simulink model "quadrotor_1d_v3"  (R2025b)
settings: Solver=ode45  StartTime=0.0  StopTime=20  MaxStep=0.005  RelTol=1e-3
values from neighbouring files (symbols this model uses):
  agr_scale = 1.4    [quad_params_v2.m]
  c_d = 0.1    [quad_params_v2.m]
  ctrl_mode = 0    [quad_params_v2.m]    (also in run_compare_v2.m)
  g = 9.81    [quad_params_v2.m]
  gamma = 0.40    (= 0.4)    [quad_params_v2.m]
  k_f = m*g/(4*w_hover^2)    (= 5.00510204082e-06)    [quad_params_v2.m]
  Kd0 = Kd    [design_pid_v2.m]
  Ki0 = Ki    [design_pid_v2.m]
  Kp0 = Kp    [design_pid_v2.m]
  m = 1.0    (= 1)    [quad_params_v2.m]
  tau_m = 0.05    [quad_params_v2.m]
  U_max = 2*m*g    (= 19.62)    [quad_params_v2.m]
  w_hover = 700    [quad_params_v2.m]
  w_max = sqrt(U_max/(4*k_f))    [quad_params_v2.m]
  wind_amp = -6.0    (= -6)    [quad_params_v2.m]
  wind_dur = 3.0    (= 3)    [quad_params_v2.m]
  wind_t0 = 5.0    (= 5)    [quad_params_v2.m]
  z0 = 0    [quad_params_v2.m]
undefined symbols (not defined in the file or in its folder): b1, b2, b3, W1, W2, W3
libraries: simulink x2
settings Model: Creator=Monster  LastModifiedBy=Monster

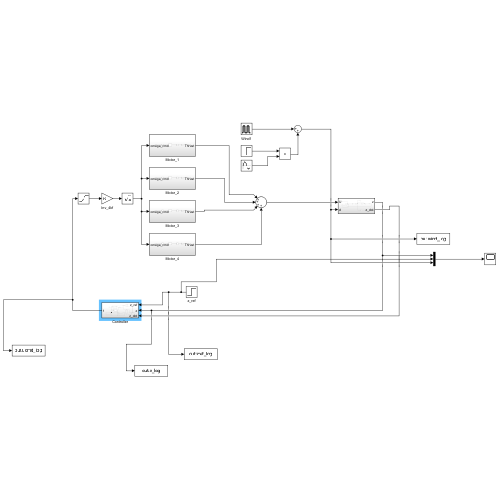
[thumbnail: Simulink's stored preview of the top-level diagram]
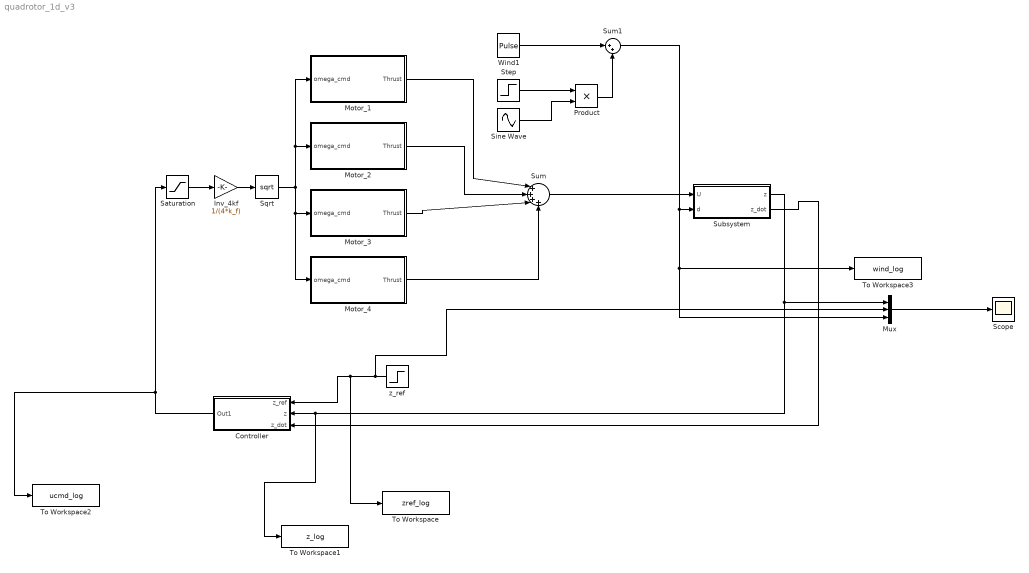
== system quadrotor_1d_v3 ==
  Controller : Subsystem
  Inv_4kf : Gain  Gain=1/(4*k_f)
  Motor_1 : Subsystem
  Motor_2 : Subsystem
  Motor_3 : Subsystem
  Motor_4 : Subsystem
  Mux : Mux  Inputs=3
  Product : Product
  Saturation : Saturate  UpperLimit=U_max  LowerLimit=0  ZeroCross=off
  Scope : Scope
      settings: ActiveDisplayYMinimum=-11.330608642093068  ActiveDisplayYMaximum=2.393195803335681
  Sine Wave : Sin  Amplitude=3  Frequency=2  Phase=-24  SampleTime=0
  Sqrt : Sqrt
  Step : Step  Time=12  SampleTime=0
  Subsystem : Subsystem
  Sum : Sum  Inputs=|++++
  Sum1 : Sum  Inputs=|++
  To Workspace : ToWorkspace  VariableName=zref_log  SampleTime=-1
  To Workspace1 : ToWorkspace  VariableName=z_log  SampleTime=-1
  To Workspace2 : ToWorkspace  VariableName=ucmd_log  SampleTime=-1
  To Workspace3 : ToWorkspace  VariableName=wind_log  SampleTime=-1
  Wind1 : DiscretePulseGenerator  PulseType=Time based  Amplitude=wind_amp  Period=20  PulseWidth=100*wind_dur/20  PhaseDelay=wind_t0
  z_ref : Step  After=0.2  SampleTime=0
  wires:
  Inv_4kf/1 -> Sqrt/1
  Controller/1(Out1) -> To Workspace2/1, Saturation/1
  Saturation/1 -> Inv_4kf/1
  Sqrt/1 -> Motor_2/1(omega_cmd), Motor_1/1(omega_cmd), Motor_4/1(omega_cmd), Motor_3/1(omega_cmd)
  Motor_1/1(Thrust) -> Sum/1
  Motor_2/1(Thrust) -> Sum/2
  Motor_3/1(Thrust) -> Sum/3
  Motor_4/1(Thrust) -> Sum/4
  Sum/1 -> Subsystem/1(U)
  Sum1/1 -> Mux/3, To Workspace3/1, Subsystem/2(d)
  Subsystem/2(z_dot) -> Controller/3(z_dot)
  Subsystem/1(z) -> To Workspace1/1, Controller/2(z), Mux/1
  Mux/1 -> Scope/1
  z_ref/1 -> Mux/2, To Workspace/1, Controller/1(z_ref)
  Sine Wave/1 -> Product/2
  Step/1 -> Product/1
  Wind1/1 -> Sum1/1
  Product/1 -> Sum1/2

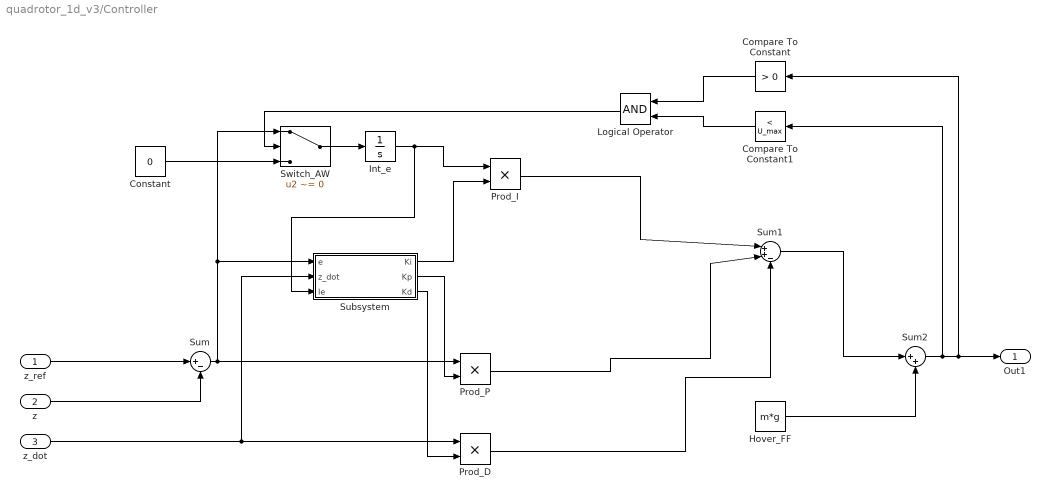
== system quadrotor_1d_v3/Controller ==
  z_ref : Inport
  z : Inport  Port=2
  z_dot : Inport  Port=3
  Compare To Constant : simulink/Logic and Bit Operations/Compare To Constant  relop=>  const=0  OutDataTypeStr=boolean  ZeroCross=off
  Compare To Constant1 : simulink/Logic and Bit Operations/Compare To Constant  relop=<  const=U_max  OutDataTypeStr=boolean
  Constant : Constant  Value=0
  Hover_FF : Constant  Value=m*g
  Int_e : Integrator
  Logical Operator : Logic  AllPortsSameDT=off  OutDataTypeStr=boolean
  Prod_D : Product
  Prod_I : Product
  Prod_P : Product
  Subsystem : Subsystem
  Sum : Sum  Inputs=|+-
  Sum1 : Sum  Inputs=|++-
  Sum2 : Sum  Inputs=|++
  Switch_AW : Switch  Criteria=u2 ~= 0  ZeroCross=off  SaturateOnIntegerOverflow=off  InputSameDT=off
  Out1 : Outport
  wires:
  z_ref/1 -> Sum/1
  z/1 -> Sum/2
  Sum/1 -> Subsystem/1(e), Switch_AW/1, Prod_P/1
  z_dot/1 -> Subsystem/2(z_dot), Prod_D/1
  Sum1/1 -> Sum2/1
  Hover_FF/1 -> Sum2/2
  Sum2/1 -> Compare To Constant1/1, Compare To Constant/1, Out1/1
  Int_e/1 -> Subsystem/3(Ie), Prod_I/1
  Constant/1 -> Switch_AW/3
  Compare To Constant/1 -> Logical Operator/1
  Compare To Constant1/1 -> Logical Operator/2
  Logical Operator/1 -> Switch_AW/2
  Switch_AW/1 -> Int_e/1
  Prod_I/1 -> Sum1/1
  Prod_P/1 -> Sum1/2
  Prod_D/1 -> Sum1/3
  Subsystem/2(Kp) -> Prod_P/2
  Subsystem/1(Ki) -> Prod_I/2
  Subsystem/3(Kd) -> Prod_D/2

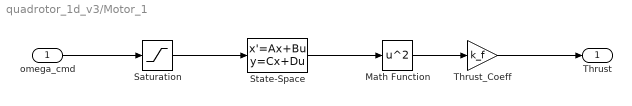
== system quadrotor_1d_v3/Motor_1 ==
  omega_cmd : Inport
  Math Function : Math  Operator=square
  Saturation : Saturate  UpperLimit=w_max  LowerLimit=0
  State-Space : StateSpace  A=-1/tau_m  B=1/tau_m  D=0  InitialCondition=w_hover
  Thrust_Coeff : Gain  Gain=k_f
  Thrust : Outport
  wires:
  Thrust_Coeff/1 -> Thrust/1
  Saturation/1 -> State-Space/1
  State-Space/1 -> Math Function/1
  Math Function/1 -> Thrust_Coeff/1
  omega_cmd/1 -> Saturation/1

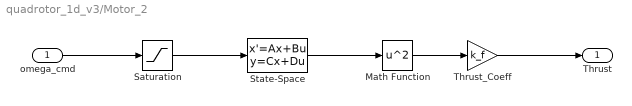
== system quadrotor_1d_v3/Motor_2 ==
  omega_cmd : Inport
  Math Function : Math  Operator=square
  Saturation : Saturate  UpperLimit=w_max  LowerLimit=0
  State-Space : StateSpace  A=-1/tau_m  B=1/tau_m  D=0  InitialCondition=w_hover
  Thrust_Coeff : Gain  Gain=k_f
  Thrust : Outport
  wires:
  Thrust_Coeff/1 -> Thrust/1
  Saturation/1 -> State-Space/1
  State-Space/1 -> Math Function/1
  Math Function/1 -> Thrust_Coeff/1
  omega_cmd/1 -> Saturation/1

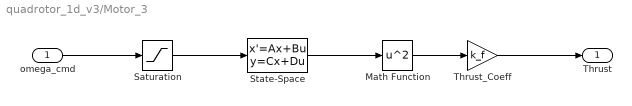
== system quadrotor_1d_v3/Motor_3 ==
  omega_cmd : Inport
  Math Function : Math  Operator=square
  Saturation : Saturate  UpperLimit=w_max  LowerLimit=0
  State-Space : StateSpace  A=-1/tau_m  B=1/tau_m  D=0  InitialCondition=w_hover
  Thrust_Coeff : Gain  Gain=k_f
  Thrust : Outport
  wires:
  Thrust_Coeff/1 -> Thrust/1
  Saturation/1 -> State-Space/1
  State-Space/1 -> Math Function/1
  Math Function/1 -> Thrust_Coeff/1
  omega_cmd/1 -> Saturation/1

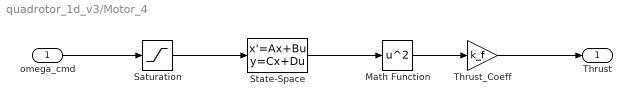
== system quadrotor_1d_v3/Motor_4 ==
  omega_cmd : Inport
  Math Function : Math  Operator=square
  Saturation : Saturate  UpperLimit=w_max  LowerLimit=0
  State-Space : StateSpace  A=-1/tau_m  B=1/tau_m  D=0  InitialCondition=w_hover
  Thrust_Coeff : Gain  Gain=k_f
  Thrust : Outport
  wires:
  Thrust_Coeff/1 -> Thrust/1
  Saturation/1 -> State-Space/1
  State-Space/1 -> Math Function/1
  Math Function/1 -> Thrust_Coeff/1
  omega_cmd/1 -> Saturation/1

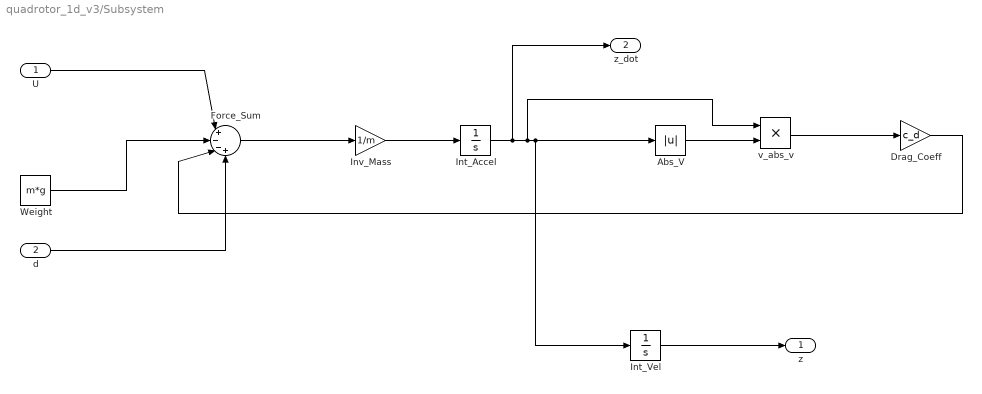
== system quadrotor_1d_v3/Subsystem ==
  U : Inport
  d : Inport  Port=2
  Abs_V : Abs  SaturateOnIntegerOverflow=off
  Drag_Coeff : Gain  Gain=c_d
  Force_Sum : Sum  Inputs=|+--+
  Int_Accel : Integrator
  Int_Vel : Integrator  InitialCondition=z0
  Inv_Mass : Gain  Gain=1/m
  Weight : Constant  Value=m*g
  v_abs_v : Product
  z : Outport
  z_dot : Outport  Port=2
  wires:
  U/1 -> Force_Sum/1
  Weight/1 -> Force_Sum/2
  d/1 -> Force_Sum/4
  Drag_Coeff/1 -> Force_Sum/3
  Force_Sum/1 -> Inv_Mass/1
  Inv_Mass/1 -> Int_Accel/1
  Int_Accel/1 -> z_dot/1, v_abs_v/1, Abs_V/1, Int_Vel/1
  Abs_V/1 -> v_abs_v/2
  v_abs_v/1 -> Drag_Coeff/1
  Int_Vel/1 -> z/1

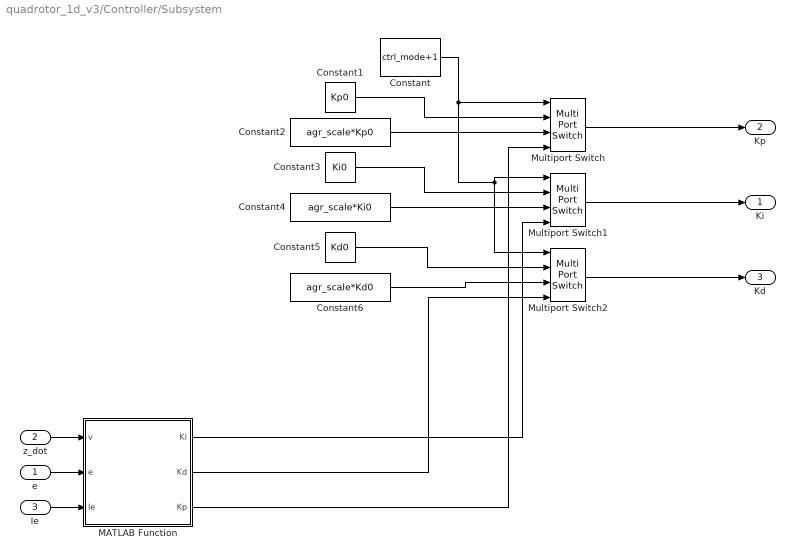
== system quadrotor_1d_v3/Controller/Subsystem ==
  e : Inport
  z_dot : Inport  Port=2
  Ie : Inport  Port=3
  Constant : Constant  Value=ctrl_mode+1
  Constant1 : Constant  Value=Kp0
  Constant2 : Constant  Value=agr_scale*Kp0
  Constant3 : Constant  Value=Ki0
  Constant4 : Constant  Value=agr_scale*Ki0
  Constant5 : Constant  Value=Kd0
  Constant6 : Constant  Value=agr_scale*Kd0
  MATLAB Function : MATLAB Function  TreatAsAtomicUnit=on
  Multiport Switch : MultiPortSwitch  SaturateOnIntegerOverflow=off  InputSameDT=off
  Multiport Switch1 : MultiPortSwitch  SaturateOnIntegerOverflow=off  InputSameDT=off
  Multiport Switch2 : MultiPortSwitch  SaturateOnIntegerOverflow=off  InputSameDT=off
  Ki : Outport
  Kp : Outport  Port=2
  Kd : Outport  Port=3
  wires:
  Constant/1 -> Multiport Switch2/1, Multiport Switch1/1, Multiport Switch/1
  Constant1/1 -> Multiport Switch/2
  Constant2/1 -> Multiport Switch/3
  Constant3/1 -> Multiport Switch1/2
  Constant4/1 -> Multiport Switch1/3
  Constant5/1 -> Multiport Switch2/2
  Constant6/1 -> Multiport Switch2/3
  Multiport Switch/1 -> Kp/1
  Multiport Switch1/1 -> Ki/1
  Multiport Switch2/1 -> Kd/1
  e/1 -> MATLAB Function/2(e)
  z_dot/1 -> MATLAB Function/1(v)
  Ie/1 -> MATLAB Function/3(Ie)
  MATLAB Function/1(Ki) -> Multiport Switch1/4
  MATLAB Function/3(Kp) -> Multiport Switch/4
  MATLAB Function/2(Kd) -> Multiport Switch2/4

== matlab function quadrotor_1d_v3/Controller/Subsystem/MATLAB Function ==
  data: W1 parameter; b1 parameter; W2 parameter; b2 parameter; W3 parameter; b3 parameter; Kp0 parameter; Ki0 parameter; Kd0 parameter; gamma parameter; v input; e input; Ie input; Ki output; Kd output; Kp output
function [Ki, Kd, Kp] = nags_pid_fcn(W1, b1, W2, b2, W3, b3, Kp0, Ki0, Kd0, gamma, v, e, Ie)
%#codegen
% Base Workspace'ten çekilenler: W1, b1, W2, b2, W3, b3, Kp0, Ki0, Kd0, gamma

% 1. Girdi Normalizasyonu
e_norm  = e / 0.5;
v_norm  = v / 2.0;
Ie_norm = Ie / 2.0;

x = [e_norm; v_norm; Ie_norm];

% 2. İleri Besleme Katmanları (ReLU)
h1 = max(0, W1 * x + b1);
h2 = max(0, W2 * h1 + b2);

% 3. Çıkış Katmanı (Tanh) ve %40 Ölçekleme
out = tanh(W3 * h2 + b3);

dKp = out(1) * gamma;
dKi = out(2) * gamma;
dKd = out(3) * gamma;

% 4. Dinamik PID Kazançları
Kp = Kp0 * (1.0 + dKp);
Ki = Ki0 * (1.0 + dKi);
Kd = Kd0 * (1.0 + dKd);
end
